simulink model "PMSMdetailTestbench"  (R2025b)
settings: Solver=ode1be  StartTime=0.0  StopTime=50  FixedStep=electricDrive.PmsmControlParams.Ts  RelTol=1e-3  EnableMultiTasking=on
PreLoadFcn:
  | PMSMSystemParams;
  | %PMSMthermalParams;
undefined symbols (not defined in the file or in its folder): electricDrive
libraries: fl_lib x91, nesl_utility x22, ee_lib x4, SimscapeFluids_lib x3, eeTransforms x2, simulink x2, batteryecm_lib x1, autolibshared x1, sdl_lib x1, eePmsmCurrentController x1, eePmsmFwController x1, eePmsmCurrentReferenceGen x1
(part 1 of 2)
CloseFcn:
  | try,close(h1_ee_pmsm_field_weakening_control),end
  | clear h1_ee_pmsm_field_weakening_control
  | 
  | clear simlogPMSMfocControlLossMaoGen
  | clear logsoutPMSMfocControlLossMaoGen
  | clear air_density alpha beta  Cdc CopperDensity CopperSpHeat CopperThconductivity Cp Cv drag_coefficient dt  gravity h h_conv IronDensity IronSpHeat IronThConductivity Jm k Ld lossMat Lq  max_power max_torque MotorThermal nu p Pmax PmsmControlParams PmsmParams rho  spMat tqMat tout T Tmax  u VehicleParams Vnom
Description:
  | Copyright 2022 - 2023 The MathWorks, Inc.
settings Model: Creator=The MathWorks, Inc.  LastModifiedBy=jjha
settings SolverCC: AlgebraicLoopSolver=TrustRegion  AutoInsertRateTranBlk=on  MaxZcPerStep=1.0
settings DataIOCC: MaxDataPoints=210000  SignalLoggingName=logsoutPMSMdetailTestbench  ReturnWorkspaceOutputsName=simoutPMSMdetailTestbench
settings OptimizationCC: ReuseModelBlockBuffer=off  LifeSpan=inf
settings DebuggingCC: UnconnectedInputMsg=warning  UnconnectedOutputMsg=warning  UnconnectedLineMsg=warning  SFUnexpectedBacktrackingDiag=warning  SFNoUnconditionalDefaultTransitionDiag=warning  SFExecutionAtInitializationDiag=none  ArithmeticOperatorsInVariantConditions=warning
settings ModelReferenceCC: EnableRefExpFcnMdlSchedulingChecks=on
settings SFSimCC: SimUseLocalCustomCode=off  CustomCodeUndefinedFunction=UseInterfaceOnly
settings RTWCC: RTWUseLocalCustomCode=off  GPUComputeCapability=3.5  DLArmComputeVersion=19.05
settings CodeAppCC: StateflowObjectComments=on
settings GRTTargetCC: TargetLangStandard=C89/C90 (ANSI)
settings ConfigComp: CovMetricSettings=dw  CovSaveCumulativeToWorkspaceVar=on  CovSaveSingleToWorkspaceVar=on  CovExternalEMLEnable=off
settings SimscapeCC: SimscapeNormalizeSystem=off  SimscapeLogType=all  SimscapeLogSimulationStatistics=on  SimscapeLogName=simlogPMSMdetailTestbench  SimscapeLogDataHistory=700000.0

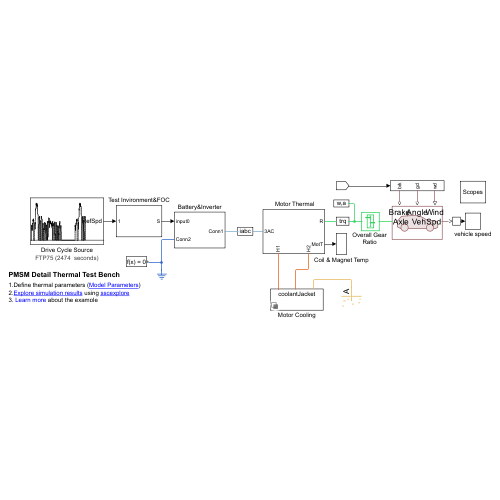
[thumbnail: Simulink's stored preview of the top-level diagram]
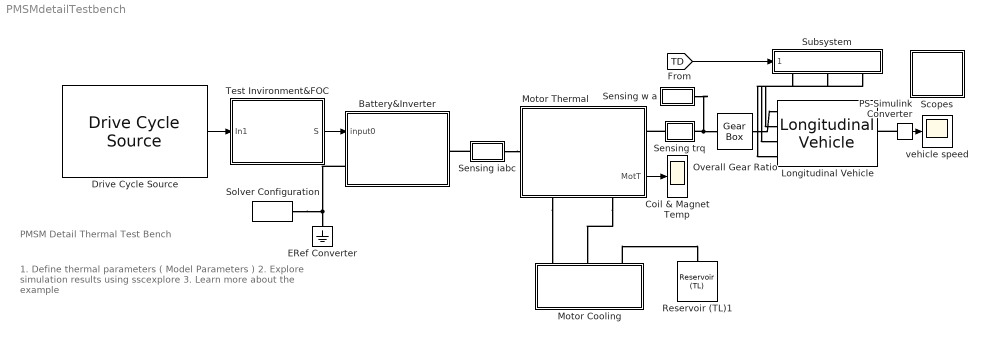
== system PMSMdetailTestbench ==
  note: PMSM Detail Thermal Test Bench
  note: 1. Define thermal parameters ( Model Parameters )
      | 2. Explore simulation results using sscexplore
      | 3. Learn more about the example
  " Motor Thermal" : Subsystem  Tag=PublishSubsystem  VariantControl=Variant1
      settings: PortSchema="{\"entries\":[{\"content\":{\"sides\":[{\"content\":{\"connectorIds\":[\"LConn1\"]},\"type\":\"ConnectorPlacement.EquallySpacedRectSide\",\"uuid\":\"590a444e-8195-4988-a9c8-7c57f93e7add\"},{\"content\":{\"connectorIds\":[\"RConn1\",\"Out1\"],\"side\":\"RIGHT\"},\"type\":\"ConnectorPlacement.EquallySpacedRectSide\",\"uuid\":\"ff30d583-60d1-4c2f-8cfa-0519d0956af2\"},{\"content\":{\"connectorIds\":[],\"side\":\"TOP\"},\"type\":\"ConnectorPlacement.EquallySpacedRectSide\",\"uuid\":\"f416ecb7-f0fa-4dcd-bce9-4bdf16786e53\"},{\"content\":{\"connectorIds\":[\"RConn2\",\"RConn3\"],\"side\":\"BOTTOM\"},\"type\":\"ConnectorPlacement.EquallySpacedRectSide\",\"uuid\":\"aeecbe3b-4b08-4b99-ab7c-25ad9565aff3\"}]},\"type\":\"ConnectorPlacement.EquallySpacedConnector\",\"uuid\":\"9ecfe474-afdb-4e00-8545-4450812d4813\"}],\"packageUris\":[\"http://schema.mathworks.com/mf0/Connector/R2020b\"],\"version\":\"1.0\"}"
  Battery&Inverter : Subsystem
  Coil & Magnet Temp : Scope
      settings: ActiveDisplayYMinimum=-45.49094  ActiveDisplayYMaximum=409.41849
  Drive Cycle Source : autolibshared/Drive Cycle Source  cycleVar=FTP75  fileVar=cycleFTP75.mat  tfinal="2474  seconds"  cycleRepeat=off  outAccPort=off  outGearPort=off  gearList=No gear data  t_wot1=5  xdot_woto=0  xdot_wot1=30  t_wot2=20  xdot_wot2=0  t_wotend=30  srcUnit=m/s  outUnit=km/hr  srcAccUnit=m/s/s  outAccUnit=m/s^2  dt=1e-3  aMode=1  faultOption=off  velBnd=2  velBndUnit=mph  inUnit=m/s  timeBnd=1  failOption=off  stopSim=off  maxFaultCnt=10  maxFaultTime=2  maxTotFaultTime=15  traceOption=off  dtTrace=1  traceWindow=10  lastDCname=FTP75  lastOutUnit=mph  lastDT=1e-3  lastTB=1  lastSB=2  forceCalcBound=off
  ERef Converter : fl_lib/Electrical/Electrical Elements/Electrical Reference
  Longitudinal Vehicle : sdl_lib/Tires & Vehicles/Longitudinal Vehicle  vehParamType=sdl.enum.VehicleParameterizationType.Regular  M_vehicle=electricDrive.VehicleParams.vehicle_mass kg  R_tireroll=electricDrive.VehicleParams.wheel_radius m  C_tireroll=electricDrive.VehicleParams.rolling_res_ratio  C_airdrag=electricDrive.drag_coefficient  A_front=electricDrive.VehicleParams.Frontalarea m^2  A_rl=120 N  B_rl=1.8 N*s/m  C_rl=0.389 N*s^2/m^2  g=electricDrive.gravity m/s^2  V_1=0.3 m/s  w_1=0.01 rad/s  ShowBrakeIn=true  ShowSlopeIn=true  SlopeInputType=sdl.enum.VehicleLongitudinalRoadSlopeInputType.Angle  ShowWindIn=true  ShowGOut=false  air_density=1.184 kg/m^3  V_x_specify=off  V_x_priority=High  V_x=0 m/s  V_x_nominal_specify=off  V_x_nominal_value=1  V_x_nominal_unit=m/s  trq_specify=off  trq_priority=None  trq=0 N*m  trq_nominal_specify=off  trq_nominal_value=1  trq_nominal_unit=N*m  w_specify=off  w_priority=None  w=0 rad/s  w_nominal_specify=off  w_nominal_value=1  w_nominal_unit=rad/s
      settings: InternalSimscapePortConfiguration="{\"Bottom\":[],\"Left\":[{\"id\":\"Axle\",\"label\":\"Axle\",\"type\":\"foundation.mechanical.rotational.rotational\"}],\"Right\":[{\"id\":\"v_out\",\"label\":\"VehSpd\",\"type\":\"output\"}],\"Top\":[{\"id\":\"brkF\",\"label\":\"Brake\",\"type\":\"input\"},{\"id\":\"angle_in\",\"label\":\"Angle\",\"type\":\"input\"},{\"id\":\"V_wind\",\"label\":\"Wind\",\"type\":\"input\"}]}"
  Motor Cooling : Subsystem  Variant=on  VariantControlMode=label  LabelModeActiveChoice=true
      settings: PortSchema="{\"entries\":[{\"content\":{\"sides\":[{\"content\":{\"connectorIds\":[]},\"type\":\"ConnectorPlacement.EquallySpacedRectSide\",\"uuid\":\"fad2e2e2-c8a8-4ae7-a5e0-e2d04801ad81\"},{\"content\":{\"connectorIds\":[],\"side\":\"RIGHT\"},\"type\":\"ConnectorPlacement.EquallySpacedRectSide\",\"uuid\":\"a876eae4-26d9-44a3-9dd3-410a35dafbf1\"},{\"content\":{\"connectorIds\":[\"LConn1\",\"LConn2\",\"LConn3\"],\"side\":\"TOP\"},\"type\":\"ConnectorPlacement.EquallySpacedRectSide\",\"uuid\":\"b2d352a8-e78b-4f23-87e4-b1c134d4f518\"}]},\"type\":\"ConnectorPlacement.EquallySpacedConnector\",\"uuid\":\"4da0a1ca-7739-4d5f-a9bc-f50bcf2d911d\"}],\"packageUris\":[\"http://schema.mathworks.com/mf0/Connector/R2020b\"],\"version\":\"1.0\"}"
  "Overall Gear Ratio " : fl_lib/Mechanical/Mechanisms/Gear Box  ratio=electricDrive.VehicleParams.Gear_ratio  t_in_specify=off  t_in_priority=High  t_in=0 N*m  t_in_nominal_specify=off  t_in_nominal_value=1  t_in_nominal_unit=N*m  t_out_specify=off  t_out_priority=High  t_out=0 N*m  t_out_nominal_specify=off  t_out_nominal_value=1  t_out_nominal_unit=N*m
  PS-Simulink Converter : nesl_utility/PS-Simulink Converter  PhysicalDomain=network_engine_domain  SubClassName=ps_output  LeftPortType=input  RightPortType=output  PseudoPeriodic=off  Frequencies=[]  VectorFormat=inherit  Unit=inherit  AffineConversion=off
  Reservoir (TL)1 : fl_lib/Thermal Liquid/Elements/Reservoir (TL)  pressure_spec=foundation.enum.pressure_spec.atmospheric  reservoir_pressure=0.101325 MPa  reservoir_temperature=293.15 K  area=0.01 m^2
  Scopes : Subsystem
      mask Display: disp(get_param(gcb,'Name'))
  Sensing w a : Subsystem
      mask Display: disp('w,a')
  Sensing iabc : Subsystem
      mask Display: disp('iabc')
  Sensing trq : Subsystem
      mask Display: disp('trq')
  Solver Configuration : nesl_utility/Solver Configuration  PhysicalDomain=network_engine_domain  SubClassName=solver  LeftPortType=input  RightPortType=generic  Tones=[]  Harmonics=[]  SimulateNoise=off  Profile=off  UseLocalSampling=off  EnableSwitchedLinearOptims=on  FrequencyDomain=off  UseCCode=off  RelTol=0.001  AbsTol=1e-06  MinStep=1e-09  ToWorkspace=off  RevertToSquareIcSolve=off  NumHomotopyIterations=100  PhasorMode=off  PhasorModeNumHarmonics=1  ConsistencySolver=NEWTON_XTOL_AFTER_FTOL  IndexReductionMethod=DerivativeReplacement  DoDC=off  ResidualTolerance=1e-9  ConsistencyTolSource=GLOBAL  ConsistencyAbsTol=0.001  ConsistencyRelTol=0.001  ConsistencyTolFactor=0.001  UseLocalSolver=on  LocalSolverChoice=NE_BACKWARD_EULER_ADVANCER  ResolveIndetEquations=on  FunctionEvalNumThread=1  LocalSolverSampleTime=electricDrive.PmsmControlParams.Ts  DoFixedCost=on  MaxNonlinIter=4  MaxModeIter=2  ComputeImpulses=off  ImpulseIterations=2  LinearAlgebra=auto  LinearAlgebraNumThread=0  EquationFormulation=NE_TIME_EF  DelaysMemoryBudget=1024  AutomaticFiltering=on  FilteringTimeConstant=0.001  PartitionStorageMethod=AS_NEEDED  PartitionMemoryBudget=1024  PartitionMethod=FAST  MultibodyUseLocalSolver=off  MultibodyLocalSolverChoice=ODE1  MultibodyLocalSolverSampleTime=0.001
  Subsystem : Subsystem
      settings: PortSchema="{\"entries\":[{\"content\":{\"sides\":[{\"content\":{\"connectorIds\":[]},\"type\":\"ConnectorPlacement.EquallySpacedRectSide\",\"uuid\":\"5b33bb33-1028-4467-9d0b-860d7c65cb16\"},{\"content\":{\"connectorIds\":[\"RConn1\",\"RConn2\",\"RConn3\"],\"side\":\"RIGHT\"},\"type\":\"ConnectorPlacement.EquallySpacedRectSide\",\"uuid\":\"d30bcb89-569c-4584-a5e8-bf96143649ac\"},{\"content\":{\"connectorIds\":[\"In1\"],\"side\":\"TOP\"},\"type\":\"ConnectorPlacement.EquallySpacedRectSide\",\"uuid\":\"a556bd16-04f6-4e3c-9a78-edea790b19fa\"}]},\"type\":\"ConnectorPlacement.EquallySpacedConnector\",\"uuid\":\"7b9502e3-af00-49d8-8813-697019fc00d4\"}],\"packageUris\":[\"http://schema.mathworks.com/mf0/Connector/R2020b\"],\"version\":\"1.0\"}"
  Test Invironment&FOC : Subsystem
  vehicle speed : Scope
      settings: ActiveDisplayYMinimum=-1.28909  ActiveDisplayYMaximum=11.51595  DataLoggingVariableName=ScopeData2
  wires:
  Drive Cycle Source/1 -> Test Invironment&FOC/1(In1)
  Test Invironment&FOC/1(S) -> Battery&Inverter/1(input0)
  [TD] -> Subsystem/1(" ")
  PS-Simulink Converter/1 -> vehicle speed/1
  " Motor Thermal"/1(MotT) -> Coil & Magnet Temp/1
  connections:
  Sensing iabc/RConn1 -- " Motor Thermal"/LConn1
  Sensing trq/LConn1 -- " Motor Thermal"/RConn1
  Sensing w a/LConn1 -- Sensing trq/RConn1 -- "Overall Gear Ratio "/LConn1
  Sensing iabc/LConn1 -- Battery&Inverter/RConn1
  Battery&Inverter/LConn1 -- Solver Configuration/RConn1 -- ERef Converter/LConn1
  Subsystem/RConn1 -- Longitudinal Vehicle/LConn2
  Subsystem/RConn2 -- Longitudinal Vehicle/LConn3
  PS-Simulink Converter/LConn1 -- Longitudinal Vehicle/RConn1
  "Overall Gear Ratio "/RConn1 -- Longitudinal Vehicle/LConn1
  Subsystem/RConn3 -- Longitudinal Vehicle/LConn4
  Motor Cooling/LConn3 -- Reservoir (TL)1/LConn1
  " Motor Thermal"/RConn3 -- Motor Cooling/LConn2
  " Motor Thermal"/RConn2 -- Motor Cooling/LConn1

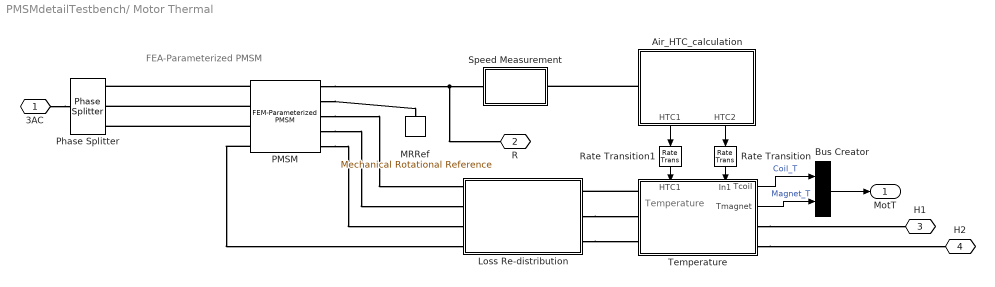
== system PMSMdetailTestbench/ Motor Thermal ==
  note: Temperature
  note: FEA-Parameterized
      | PMSM
  Air_HTC_calculation : Subsystem
      settings: PortSchema="{\"entries\":[{\"content\":{\"sides\":[{\"content\":{\"connectorIds\":[\"LConn1\"]},\"type\":\"ConnectorPlacement.EquallySpacedRectSide\",\"uuid\":\"c3fc49c2-0151-484f-b0d8-f4e4a060bcaf\"},{\"content\":{\"side\":\"RIGHT\"},\"type\":\"ConnectorPlacement.EquallySpacedRectSide\",\"uuid\":\"c73251fe-fcad-4c5f-9d27-fb7ac98c9b31\"},{\"content\":{\"side\":\"TOP\"},\"type\":\"ConnectorPlacement.EquallySpacedRectSide\",\"uuid\":\"06ea8515-c1b4-4445-9ea2-9a6fe3b8d822\"},{\"content\":{\"connectorIds\":[\"Out1\",\"Out2\"],\"side\":\"BOTTOM\"},\"type\":\"ConnectorPlacement.EquallySpacedRectSide\",\"uuid\":\"0d77474d-64a7-49ab-b2b5-eb3962b26dfa\"}]},\"type\":\"ConnectorPlacement.EquallySpacedConnector\",\"uuid\":\"651eda7a-2416-4496-9b8b-1b2d725cf6dd\"}],\"packageUris\":[\"http://schema.mathworks.com/mf0/Connector/R2020b\"],\"version\":\"1.0\"}"
  Bus Creator : BusCreator  Inputs=2
  Loss Re-distribution : Subsystem
  MRRef : fl_lib/Mechanical/Rotational Elements/Mechanical Rotational Reference
  PMSM : ee_lib/Electromechanical/Permanent Magnet/FEM-Parameterized PMSM  parameterization=1  winding_type=ee.enum.statorconnection.wye  iVec=[-2, 0, 2] A  xVec=[0, 20, 40, 60] deg  dfluxdiMatrix=0.0002 * ones(3, 4) Wb/A  dfluxdxMatrix=[0, -.16, .16, 0; 0, -.16, .16, 0; 0, -.16, .16, 0] Wb/rad  calculate_torque_matrix=1  TorqueMatrix=zeros(3, 3, 3, 4) N*m  idVec1=[-200, 0, 200] A  iqVec1=[-200, 0, 200] A  LdMatrix=0.0002 * ones(3, 3) H  LqMatrix=0.0002 * ones(3, 3) H  PmMatrix=0.1 * ones(3, 3) Wb  interp_method=simscape.enum.interpolation.linear  N=6  Rs=electricDrive.PmsmParams.StatorResistance Ohm  Ms=0.00002 H  L0=0.00016 H  loss_param=ee.enum.fem_motor.ironLossesExtended.tabulated  losses_oc=[0, 0, 0] W  losses_sc=[0, 0, 0] W  f_losses=100 % dummy value, not required Hz  Isc_losses=95 A  Inertia=electricDrive.PmsmParams.RotorInertia kg*m^2  lam=0 N*m/(rad/s)  i_d_specify=off  i_d_priority=High  i_d=0 A  i_d_nominal_specify=off  i_d_nominal_value=1  i_d_nominal_unit=A  i_q_specify=off  i_q_priority=High  i_q=0 A  i_q_nominal_specify=off  i_q_nominal_value=1  i_q_nominal_unit=A  torque_specify=off  torque_priority=None  torque=0 N*m  torque_nominal_specify=off  torque_nominal_value=1  torque_nominal_unit=N*m  angular_velocity_specify=off  angular_velocity_priority=High  angular_velocity=PmsmParams.InitialRotorSpeed_rpm rpm  angular_velocity_nominal_specify=off  angular_velocity_nominal_value=1  angular_velocity_nominal_unit=rpm  angular_position_specify=on  angular_position_priority=High  angular_position=electricDrive.PmsmParams.InitialRotorAngle_rad rad  angular_position_nominal_specify=off  angular_position_nominal_value=1  angular_position_nominal_unit=deg  alpha=0.00386 1/K  alpha_flux=-0.001 1/K  Tmeas=283.15 K  stator_thermal_mass=electricDrive.MotorThermal.PhaseWindingThMass J/K  stator_initial_temperatures=[298.15, 298.15, 298.15] K  rotor_thermal_mass=electricDrive.MotorThermal.RotorThMass J/K  rotor_initial_temperature=298.15 K  Rm_percent_rotor=90  Rd_percent_rotor=30  idVec=[-200, 0, 200] A  iqVec=[-200, 0, 200] A  dfluxAdiaMatrix3D=zeros(3, 3, 4) Wb/A  dfluxAdibMatrix3D=zeros(3, 3, 4) Wb/A  dfluxAdicMatrix3D=zeros(3, 3, 4) Wb/A  dfluxAdxMatrix3D=zeros(3, 3, 4) Wb/rad  TorqueMatrix3D=zeros(3, 3, 4) N*m  iaVec=[-200, 0, 200] A  ibVec=[-200, 0, 200] A  icVec=[-200, 0, 200] A  dfluxAdiaMatrix=zeros(3, 3, 3, 4) Wb/A  dfluxAdibMatrix=zeros(3, 3, 3, 4) Wb/A  dfluxAdicMatrix=zeros(3, 3, 3, 4) Wb/A  dfluxAdxMatrix=zeros(3, 3, 3, 4) Wb/rad  param_dq0=ee.enum.fem_motor.fluxTabulationOption.DQpolar  winding_type_dq0=ee.enum.statorconnection.wye  expose_neutral_port=ee.enum.fem_motor.exposeNeutralPort.no  nPolePairs=electricDrive.PmsmParams.NumPolePairs  parks_type=ee.enum.fem_motor.parksType.QleadsD_AphaseToQaxis  idVec2=[-200, 0, 200] A  iqVec2=[-200, 0, 200] A  magVec2=electricDrive.PmsmParams.CurrMagVec*1.3 A  betaVec2=electricDrive.PmsmParams.CurrAdvAngleVec deg  xVec2=electricDrive.PmsmParams.RotorAngleVec deg  fluxD_dq0=zeros(3, 3, 7) Wb  fluxQ_dq0=zeros(3, 3, 7) Wb  fluxA_dq0=zeros(3, 3, 7) Wb  Torque_dq0=zeros(3, 3, 7) N*m  fluxD_IBX=electricDrive.PmsmParams.FluxDMat Wb  fluxQ_IBX=electricDrive.PmsmParams.FluxQMat Wb  fluxA_IBX=fluxAmat Wb  Torque_IBX=electricDrive.PmsmParams.TorqueMat N*m  rotorLossCoeff_k_h_DQ=zeros(3, 3) W/Hz  rotorLossCoeff_k_J_DQ=zeros(3, 3) W/Hz^2  rotorLossCoeff_k_ex_DQ=zeros(3, 3) W/Hz^(3/2)  rotorLossCoeff_k_h_IB=electricDrive.PmsmParams.RotorKhMat W/Hz  rotorLossCoeff_k_J_IB=electricDrive.PmsmParams.RotorKjMat W/Hz^2  rotorLossCoeff_k_ex_IB=electricDrive.PmsmParams.RotorKexMat W/Hz^(3/2)  statorLossCoeff_k_h_DQ=zeros(3, 3) W/Hz  statorLossCoeff_k_J_DQ=zeros(3, 3) W/Hz^2  statorLossCoeff_k_ex_DQ=zeros(3, 3) W/Hz^(3/2)  statorLossCoeff_k_h_IB=electricDrive.PmsmParams.StatorKhMat W/Hz  statorLossCoeff_k_J_IB=electricDrive.PmsmParams.StatorKjMat W/Hz^2  statorLossCoeff_k_ex_IB=electricDrive.PmsmParams.StatorKexMat W/Hz^(3/2)  wVec=[1000, 2000] rpm  rotorLossTable_DQ=zeros(3, 3, 2) W  statorLossTable_DQ=zeros(3, 3, 2) W  rotorLossTable_IB=zeros(3, 5, 2) W  statorLossTable_IB=zeros(3, 5, 2) W  electrical_torque_before_iron_losses_specify=off  electrical_torque_before_iron_losses_priority=None  electrical_torque_before_iron_losses=0 N*m  electrical_torque_before_iron_losses_nominal_specify=off  electrical_torque_before_iron_losses_nominal_value=1  electrical_torque_before_iron_losses_nominal_unit=N*m  Qrotor_specify=off  Qrotor_priority=None  Qrotor=0 J/s  Qrotor_nominal_specify=off  Qrotor_nominal_value=1  Qrotor_nominal_unit=J/s  Qstator_specify=off  Qstator_priority=None  Qstator=0 J/s  Qstator_nominal_specify=off  Qstator_nominal_value=1  Qstator_nominal_unit=J/s
      settings: InternalSimscapePortConfiguration="{\"Bottom\":[],\"Left\":[{\"id\":\"a\",\"label\":\"a\",\"type\":\"foundation.electrical.electrical\"},{\"id\":\"b\",\"label\":\"b\",\"type\":\"foundation.electrical.electrical\"},{\"id\":\"c\",\"label\":\"c\",\"type\":\"foundation.electrical.electrical\"},{\"id\":\"HR\",\"label\":\"HR\",\"type\":\"foundation.thermal.thermal\"}],\"Right\":[{\"id\":\"R\",\"label\":\"R\",\"type\":\"foundation.mechanical.rotational.rotational\"},{\"id\":\"C\",\"label\":\"C\",\"type\":\"foundation.mechanical.rotational.rotational\"},{\"id\":\"HA\",\"label\":\"HA\",\"type\":\"foundation.thermal.thermal\"},{\"id\":\"HB\",\"label\":\"HB\",\"type\":\"foundation.thermal.thermal\"},{\"id\":\"HC\",\"label\":\"HC\",\"type\":\"foundation.thermal.thermal\"}],\"Top\":[]}"
  Phase Splitter : ee_lib/Connectors & References/Phase Splitter
  Rate Transition : RateTransition
  Rate Transition1 : RateTransition
  Speed Measurement : Subsystem
  Temperature : Subsystem
      settings: PortSchema="{\"entries\":[{\"content\":{\"sides\":[{\"content\":{\"connectorIds\":[\"LConn1\",\"LConn2\",\"LConn3\"]},\"type\":\"ConnectorPlacement.EquallySpacedRectSide\",\"uuid\":\"fee72484-960d-4cd4-9296-e38678962aa1\"},{\"content\":{\"connectorIds\":[\"Out1\",\"Out2\",\"RConn1\",\"RConn2\"],\"side\":\"RIGHT\"},\"type\":\"ConnectorPlacement.EquallySpacedRectSide\",\"uuid\":\"5fc115b4-63fd-47d3-871d-1c82ac52ac43\"},{\"content\":{\"connectorIds\":[\"In1\",\"In2\"],\"side\":\"TOP\"},\"type\":\"ConnectorPlacement.EquallySpacedRectSide\",\"uuid\":\"406f719a-f995-4122-9f35-24e8332a2e84\"},{\"content\":{\"connectorIds\":[],\"side\":\"BOTTOM\"},\"type\":\"ConnectorPlacement.EquallySpacedRectSide\",\"uuid\":\"14dc85e6-8157-4b38-8651-862ce77721cd\"}]},\"type\":\"ConnectorPlacement.EquallySpacedConnector\",\"uuid\":\"1dcc2b5d-90fd-40de-873d-99118eb86bdd\"}],\"packageUris\":[\"http://schema.mathworks.com/mf0/Connector/R2020b\"],\"version\":\"1.0\"}"
  3AC : PMIOPort  Side=Left
  R : PMIOPort  Port=2  Side=Right
  H1 : PMIOPort  Port=3  Side=Right
  H2 : PMIOPort  Port=4  Side=Right
  MotT : Outport
  wires:
  Temperature/2(Tmagnet) -> Bus Creator/2  "Magnet_T"
  Rate Transition/1 -> Temperature/2(In1)
  Air_HTC_calculation/2(HTC2) -> Rate Transition/1
  Air_HTC_calculation/1(HTC1) -> Rate Transition1/1
  Rate Transition1/1 -> Temperature/1(HTC1)
  Bus Creator/1 -> MotT/1
  Temperature/1(Tcoil) -> Bus Creator/1  "Coil_T"
  connections:
  PMSM/LConn2 -- Phase Splitter/RConn2
  PMSM/RConn2 -- MRRef/LConn1
  PMSM/RConn1 -- R/RConn1 -- Speed Measurement/LConn1
  PMSM/LConn1 -- Phase Splitter/RConn1
  Air_HTC_calculation/LConn1 -- Speed Measurement/RConn1
  Loss Re-distribution/RConn2 -- Temperature/LConn2
  Loss Re-distribution/RConn3 -- Temperature/LConn3
  PMSM/LConn3 -- Phase Splitter/RConn3
  PMSM/LConn4 -- Loss Re-distribution/LConn4
  PMSM/RConn3 -- Loss Re-distribution/LConn1
  PMSM/RConn4 -- Loss Re-distribution/LConn2
  PMSM/RConn5 -- Loss Re-distribution/LConn3
  3AC/RConn1 -- Phase Splitter/LConn1
  Temperature/LConn1 -- Loss Re-distribution/RConn1
  Temperature/RConn1 -- H1/RConn1
  Temperature/RConn2 -- H2/RConn1

== system PMSMdetailTestbench/Battery&Inverter ==
  input0 : Inport
  Average-Value Voltage Source Converter (Three-Phase) : ee_lib/Semiconductors & Converters/Converters/Average-Value Voltage Source Converter (Three-Phase)  port_option=ee.enum.threePhasePort.composite  frequency_option=ee.enum.converters.frequency.variable  input_option=ee.enum.converters.inputOption.ModWave  FRated=60 Hz  losses_parameterization=ee.enum.converters.losses.fixed  Pfixed=1 W  ks=0.01  kc1=1.7 V  kc2=0.01 Ohm  Ploss_vect=[100, 800, 1870, 3250, 4900] W  Irms_vect=[10, 100, 200, 300, 400] A  Vdc_nom=300 V  thermal_mass=30000 J/K  temperature_specify=off  temperature_priority=High  temperature=298.15 K  temperature_nominal_specify=off  temperature_nominal_value=1  temperature_nominal_unit=K
      settings: InternalSimscapePortConfiguration="{\"Bottom\":[],\"Left\":[{\"id\":\"ModWave\",\"label\":\"ModWave\",\"type\":\"input\"},{\"id\":\"N\",\"label\":\"~\",\"type\":\"foundation.electrical.three_phase\"}],\"Right\":[{\"id\":\"p\",\"label\":\"+\",\"type\":\"foundation.electrical.electrical\"},{\"id\":\"n\",\"label\":\"-\",\"type\":\"foundation.electrical.electrical\"}],\"Top\":[]}"
  Battery : batteryecm_lib/Battery  Vnom=electricDrive.Vnom V  prm_dir=1  R1_dis=2 Ohm  R1_ch=2 Ohm  R1=0.001 Ohm  prm_AH=simscape.enum.battery.prm_AH.infinite  AH=200 hr*A  V1=290 V  AH1=50 hr*A  prm_R2=1  R2=2000 Ohm  Tmeas=298.15 K  charge_measurement_port=simscape.enum.battery.enable.no  prm_dyn=1  Rp1=0.005 Ohm  tau1=30 s  Rp2=0.005 Ohm  tau2=30 s  Rp3=0.005 Ohm  tau3=30 s  Rp4=0.005 Ohm  tau4=30 s  Rp5=0.005 Ohm  tau5=30 s  prm_fade=1  N_fade=100  AH_fade=45 hr*A  R1_fade=2.02 Ohm  R1_ch_fade=2.02 Ohm  V1_fade=10.35 V  prm_age=1  prm_age_OCV=1  OCV_age=0.9  SOC_age=60  Tmeas_age=298.15 K  delta_time_age_vec=[0] d  temperature_age_vec=[273] K  OCV_scaling_age=2.2134e6  OCV_offset_age=1.632e6  temp_exp_age=0.515833569 V  t_exp_age=0.75  Vnom_T2=12 V  R1_T2=2.2 Ohm  R1_T2_dis=2.2 Ohm  R1_T2_ch=2.2 Ohm  V1_T2=11.4 V  R2_T2=2200 Ohm  Rp1_T2=0.005 Ohm  tau1_T2=30 s  Rp2_T2=0.005 Ohm  tau2_T2=30 s  Rp3_T2=0.005 Ohm  tau3_T2=30 s  Rp4_T2=0.005 Ohm  tau4_T2=30 s  Rp5_T2=0.005 Ohm  tau5_T2=30 s  Tmeas2=273.15 K  thermal_port=simscape.enum.thermaleffects.omit  thermal_mass=30000 J/K  i_specify=off  i_priority=None  i=0 A  i_nominal_specify=off  i_nominal_value=1  i_nominal_unit=A  v_specify=off  v_priority=None  v=0 V  v_nominal_specify=off  v_nominal_value=1  v_nominal_unit=V  charge_specify=on  charge_priority=High  charge=200 hr*A  charge_nominal_specify=off  charge_nominal_value=1  charge_nominal_unit=A*hr  num_cycles_specify=off  num_cycles_priority=High  num_cycles=0  num_cycles_nominal_specify=off  num_cycles_nominal_value=1  num_cycles_nominal_unit=1  temperature_specify=off  temperature_priority=High  temperature=298.15 K  temperature_nominal_specify=off  temperature_nominal_value=1  temperature_nominal_unit=K
  C : fl_lib/Electrical/Electrical Elements/Capacitor  c=electricDrive.Cdc F  r=1e-6 Ohm  g=0 1/Ohm  i_specify=off  i_priority=None  i=0 A  i_nominal_specify=off  i_nominal_value=1  i_nominal_unit=A  v_specify=off  v_priority=None  v=0 V  v_nominal_specify=off  v_nominal_value=1  v_nominal_unit=V  vc_specify=on  vc_priority=None  vc=electricDrive.Vnom V  vc_nominal_specify=off  vc_nominal_value=1  vc_nominal_unit=V
  Sensing Vdc : Subsystem
      mask Display: disp('vdc')
  Simulink-PS Converter : nesl_utility/Simulink-PS Converter  PhysicalDomain=network_engine_domain  SubClassName=ps_input  LeftPortType=input  RightPortType=output  PseudoPeriodic=off  Frequencies=[]  NoiseDistribution=none  NoiseParameters=[]  Unit=1  AffineConversion=off  FilteringAndDerivatives=provide  SimscapeFilterOrder=1  InputFilterTimeConstant=0.001  UdotUserProvided=0
  Conn2 : PMIOPort  Side=Left
  Conn1 : PMIOPort  Port=2  Side=Right
  wires:
  input0/1 -> Simulink-PS Converter/1
  connections:
  Conn1/RConn1 -- Average-Value Voltage Source Converter (Three-Phase)/LConn2
  Battery/RConn1 -- Average-Value Voltage Source Converter (Three-Phase)/RConn2 -- Sensing Vdc/RConn1 -- C/RConn1 -- Conn2/RConn1
  Sensing Vdc/LConn1 -- Average-Value Voltage Source Converter (Three-Phase)/RConn1 -- Battery/LConn1 -- C/LConn1
  Simulink-PS Converter/RConn1 -- Average-Value Voltage Source Converter (Three-Phase)/LConn1

== system PMSMdetailTestbench/Motor Cooling ==
  OilJet : Subsystem  VariantControl=false
  coolantJacket : Subsystem  VariantControl=true
  MHD : PMIOPort  Side=Left
  MHJ : PMIOPort  Port=2  Side=Left
  Ref : PMIOPort  Port=3  Side=Left

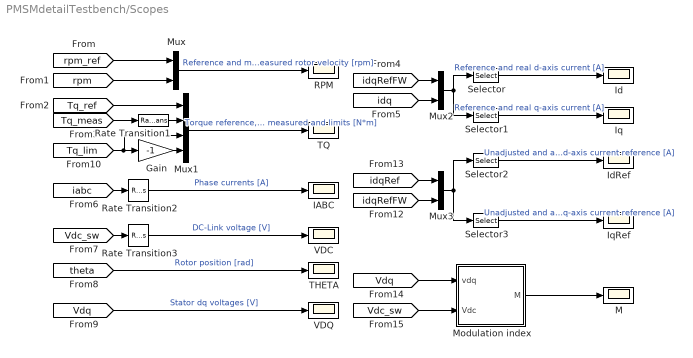
== system PMSMdetailTestbench/Scopes ==
  Gain : Gain  Gain=-1
  IABC : Scope
      settings: ActiveDisplayYMinimum=-158.01349  ActiveDisplayYMaximum=157.98632  DataLoggingSaveFormat=Array
  Id : Scope
      settings: ActiveDisplayYMinimum=-866.72955  ActiveDisplayYMaximum=3832.58854  DataLoggingVariableName=ScopeData2  DataLoggingSaveFormat=Array
  IdRef : Scope
      settings: ActiveDisplayYMinimum=-62.93355  ActiveDisplayYMaximum=6.99262  DataLoggingSaveFormat=Array
  Iq : Scope
      settings: ActiveDisplayYMinimum=-174.06811  ActiveDisplayYMaximum=31.34852  DataLoggingVariableName=ScopeData3  DataLoggingSaveFormat=Array
  IqRef : Scope
      settings: ActiveDisplayYMinimum=-26.50204  ActiveDisplayYMaximum=238.51833  DataLoggingVariableName=ScopeData2  DataLoggingSaveFormat=Array
  M : Scope
      settings: ActiveDisplayYMinimum=-0.125  ActiveDisplayYMaximum=1.125  DataLoggingSaveFormat=Array
  Modulation index : Subsystem
  Mux : Mux  Inputs=2
  Mux1 : Mux
  Mux2 : Mux  Inputs=2
  Mux3 : Mux  Inputs=2
  RPM : Scope
      settings: ActiveDisplayYMinimum=-255.1589  ActiveDisplayYMaximum=2279.13776  DataLoggingVariableName=ScopeData5  DataLoggingSaveFormat=Array
  Rate Transition1 : RateTransition
  Rate Transition2 : RateTransition  OutPortSampleTime=1e-4
  Rate Transition3 : RateTransition  OutPortSampleTime=1e-4
  Selector : Selector  InputPortWidth=4  IndexOptions=Index vector (dialog)  Indices=[1 3]  OutputSizes=1
  Selector1 : Selector  InputPortWidth=4  IndexOptions=Index vector (dialog)  Indices=[2 4]  OutputSizes=1
  Selector2 : Selector  InputPortWidth=4  IndexOptions=Index vector (dialog)  Indices=[1 3]  OutputSizes=1
  Selector3 : Selector  InputPortWidth=4  IndexOptions=Index vector (dialog)  Indices=[2 4]  OutputSizes=1
  THETA : Scope
      settings: ActiveDisplayYMinimum=-0.7854  ActiveDisplayYMaximum=7.06858  DataLoggingVariableName=ScopeData6  DataLoggingSaveFormat=Array
  TQ : Scope
      settings: ActiveDisplayYMinimum=-225.00956  ActiveDisplayYMaximum=225.00956  DataLoggingVariableName=ScopeData7  DataLoggingSaveFormat=Array
  VDC : Scope
      settings: ActiveDisplayYMinimum=-40.62138  ActiveDisplayYMaximum=365.62458  DataLoggingVariableName=ScopeData8  DataLoggingSaveFormat=Array
  VDQ : Scope
      settings: ActiveDisplayYMinimum=-210.3278  ActiveDisplayYMaximum=170.36527  DataLoggingSaveFormat=Array
  wires:
  [rpm] -> Mux/2
  Selector1/1 -> Iq/1  "Reference and real q-axis current [A]"
  Mux2/1 -> Selector1/1, Selector/1
  Gain/1 -> Mux1/4
  Rate Transition3/1 -> VDC/1  "DC-Link voltage [V]"
  [Vdc_sw] -> Rate Transition3/1
  [idqRefFW] -> Mux2/1
  [Tq_ref] -> Mux1/1
  Rate Transition2/1 -> IABC/1  "Phase currents [A]"
  [idq] -> Mux2/2
  [rpm_ref] -> Mux/1
  [iabc] -> Rate Transition2/1
  [Tq_meas] -> Rate Transition1/1
  [Vdq] -> VDQ/1  "Stator dq voltages [V]"
  Selector/1 -> Id/1  "Reference and real d-axis current [A]"
  [Tq_lim] -> Mux1/3, Gain/1
  Mux1/1 -> TQ/1  "Torque reference, measured and limits [N*m]"
  [theta] -> THETA/1  "Rotor position [rad]"
  Rate Transition1/1 -> Mux1/2
  Mux/1 -> RPM/1  "Reference and measured rotor velocity [rpm]"
  Selector2/1 -> IdRef/1  "Unadjusted and adjusted d-axis current reference [A]"
  Mux3/1 -> Selector2/1, Selector3/1
  Selector3/1 -> IqRef/1  "Unadjusted and adjusted q-axis current reference [A]"
  [idqRefFW] -> Mux3/2
  [idqRef] -> Mux3/1
  [Vdq] -> Modulation index/1(vdq)
  [Vdc_sw] -> Modulation index/2(Vdc)
  Modulation index/1(M) -> M/1

== system PMSMdetailTestbench/Sensing w a ==
  MRRef : fl_lib/Mechanical/Rotational Elements/Mechanical Rotational Reference
  Motion Sensor : fl_lib/Mechanical/Mechanical Sensors/Ideal Rotational Motion Sensor  reference=foundation.enum.MeasurementReference.difference  acceleration_port=false  velocity_port=true  position_port=true  wrap_angle=simscape.enum.onoff.off  offset=0 deg
  PS-Simulink Converter1 : nesl_utility/PS-Simulink Converter  PhysicalDomain=network_engine_domain  SubClassName=ps_output  LeftPortType=input  RightPortType=output  PseudoPeriodic=off  Frequencies=[]  VectorFormat=1-D array  Unit=rad/s  AffineConversion=off
  PS-Simulink Converter2 : nesl_utility/PS-Simulink Converter  PhysicalDomain=network_engine_domain  SubClassName=ps_output  LeftPortType=input  RightPortType=output  PseudoPeriodic=off  Frequencies=[]  VectorFormat=1-D array  Unit=rad  AffineConversion=off
  R : PMIOPort  Side=Left
  tag scope: a=global, w=global
  wires:
  PS-Simulink Converter1/1 -> [w]
  PS-Simulink Converter2/1 -> [a]
  connections:
  R/RConn1 -- Motion Sensor/LConn1
  Motion Sensor/RConn2 -- PS-Simulink Converter1/LConn1
  MRRef/LConn1 -- Motion Sensor/RConn1
  Motion Sensor/RConn3 -- PS-Simulink Converter2/LConn1

== system PMSMdetailTestbench/Sensing iabc ==
  Current Sensor : ee_lib/Sensors & Transducers/Current Sensor (Three-Phase)
  PS-Simulink Converter : nesl_utility/PS-Simulink Converter  PhysicalDomain=network_engine_domain  SubClassName=ps_output  LeftPortType=input  RightPortType=output  PseudoPeriodic=off  Frequencies=[]  VectorFormat=1-D array  Unit=A  AffineConversion=off
  1 : PMIOPort  Side=Left
  2 : PMIOPort  Port=2  Side=Right
  tag scope: iabc=global
  wires:
  PS-Simulink Converter/1 -> [iabc]
  connections:
  1/RConn1 -- Current Sensor/LConn1
  2/RConn1 -- Current Sensor/RConn2
  Current Sensor/RConn1 -- PS-Simulink Converter/LConn1

== system PMSMdetailTestbench/Sensing trq ==
  PS-Simulink Converter3 : nesl_utility/PS-Simulink Converter  PhysicalDomain=network_engine_domain  SubClassName=ps_output  LeftPortType=input  RightPortType=output  PseudoPeriodic=off  Frequencies=[]  VectorFormat=1-D array  Unit=N*m  AffineConversion=off
  Torque Sensor : fl_lib/Mechanical/Mechanical Sensors/Ideal Torque Sensor
  R : PMIOPort  Side=Left
  C : PMIOPort  Port=2  Side=Right
  tag scope: Tq_meas=global
  wires:
  PS-Simulink Converter3/1 -> [Tq_meas]
  connections:
  Torque Sensor/RConn1 -- C/RConn1
  Torque Sensor/RConn2 -- PS-Simulink Converter3/LConn1
  Torque Sensor/LConn1 -- R/RConn1

== system PMSMdetailTestbench/Subsystem ==
  " " : Inport
  Bus Selector : BusSelector  OutputSignals=Brake pedal,Incline,Wind speed
  PS Gain : fl_lib/Physical Signals/Functions/PS Gain  gain=70 N
  Simulink-PS Converter1 : nesl_utility/Simulink-PS Converter  PhysicalDomain=network_engine_domain  SubClassName=ps_input  LeftPortType=input  RightPortType=output  PseudoPeriodic=off  Frequencies=[]  NoiseDistribution=none  NoiseParameters=[]  Unit=1  AffineConversion=off  FilteringAndDerivatives=provide  SimscapeFilterOrder=1  InputFilterTimeConstant=0.001  UdotUserProvided=0
  Simulink-PS Converter2 : nesl_utility/Simulink-PS Converter  PhysicalDomain=network_engine_domain  SubClassName=ps_input  LeftPortType=input  RightPortType=output  PseudoPeriodic=off  Frequencies=[]  NoiseDistribution=none  NoiseParameters=[]  Unit=deg  AffineConversion=off  FilteringAndDerivatives=provide  SimscapeFilterOrder=1  InputFilterTimeConstant=0.001  UdotUserProvided=0
  Simulink-PS Converter3 : nesl_utility/Simulink-PS Converter  PhysicalDomain=network_engine_domain  SubClassName=ps_input  LeftPortType=input  RightPortType=output  PseudoPeriodic=off  Frequencies=[]  NoiseDistribution=none  NoiseParameters=[]  Unit=m/s  AffineConversion=off  FilteringAndDerivatives=provide  SimscapeFilterOrder=1  InputFilterTimeConstant=0.001  UdotUserProvided=0
  brk : PMIOPort  Side=Right
  gd : PMIOPort  Port=2  Side=Right
  wd : PMIOPort  Port=3  Side=Right
  wires:
  Bus Selector/2 -> Simulink-PS Converter2/1  "<Incline>"
  Bus Selector/3 -> Simulink-PS Converter3/1  "<Wind speed>"
  Bus Selector/1 -> Simulink-PS Converter1/1  "<Brake pedal>"
  " "/1 -> Bus Selector/1
  connections:
  Simulink-PS Converter2/RConn1 -- gd/RConn1
  PS Gain/RConn1 -- brk/RConn1
  Simulink-PS Converter1/RConn1 -- PS Gain/LConn1
  Simulink-PS Converter3/RConn1 -- wd/RConn1

== system PMSMdetailTestbench/Test Invironment&FOC ==
  In1 : Inport
  Field Weakning FOC Control : Subsystem
  Motor Speed Reference : Subsystem
  RT : RateTransition  OutPortSampleTime=5e-05
  Test Environment : Subsystem
  Transfer Fcn First Order : simulink/Discrete/Transfer Fcn First Order  PoleZ=0.95  ICPrevOutput=0.0  DoSatur=off
  Unit Delay : UnitDelay  SampleTime=-1  HasFrameUpgradeWarning=on
  S : Outport
  tag scope: TD=global
  wires:
  [Vdc] -> Field Weakning FOC Control/5(vdc_sens)
  In1/1 -> Unit Delay/1, RT/1
  [w] -> Field Weakning FOC Control/3(w_sens)
  [iabc] -> Field Weakning FOC Control/2(iabc_sens)
  Transfer Fcn First Order/1 -> Test Environment/1(In1)
  [a] -> Field Weakning FOC Control/4(th_sens)
  Motor Speed Reference/1(MotorSpdRef) -> Field Weakning FOC Control/1(RPMReq)
  Unit Delay/1 -> Motor Speed Reference/1(VehSpd)
  RT/1 -> Transfer Fcn First Order/1
  Test Environment/1(b) -> [TD]
  Field Weakning FOC Control/1(S) -> S/1

== system PMSMdetailTestbench/ Motor Thermal/Air_HTC_calculation ==
  Rotor side  HTC : Subsystem
  Rotor_Taylor_Couette  HTC : Subsystem
  RPM : PMIOPort  Side=Left
  HTC1 : Outport
  HTC2 : Outport  Port=2
  wires:
  Rotor side  HTC/1(Output) -> HTC2/1
  Rotor_Taylor_Couette  HTC/1(Output) -> HTC1/1
  connections:
  Rotor side  HTC/LConn1 -- RPM/RConn1 -- Rotor_Taylor_Couette  HTC/LConn1

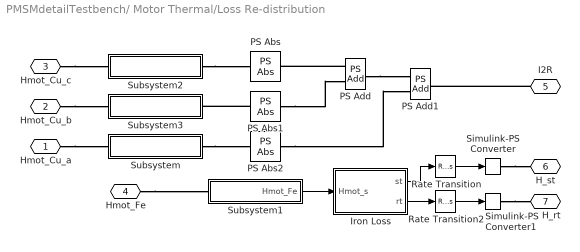
== system PMSMdetailTestbench/ Motor Thermal/Loss Re-distribution ==
  Iron Loss : Subsystem
  PS Abs : fl_lib/Physical Signals/Nonlinear Operators/PS Abs  ZeroCross=true
      settings: InternalSimscapePortConfiguration="{\"Bottom\":[],\"Left\":[{\"id\":\"I\",\"label\":\"\",\"type\":\"input\"}],\"Right\":[{\"id\":\"O\",\"label\":\"\",\"type\":\"output\"}],\"Top\":[]}"
  PS Abs1 : fl_lib/Physical Signals/Nonlinear Operators/PS Abs  ZeroCross=true
      settings: InternalSimscapePortConfiguration="{\"Bottom\":[],\"Left\":[{\"id\":\"I\",\"label\":\"\",\"type\":\"input\"}],\"Right\":[{\"id\":\"O\",\"label\":\"\",\"type\":\"output\"}],\"Top\":[]}"
  PS Abs2 : fl_lib/Physical Signals/Nonlinear Operators/PS Abs  ZeroCross=true
      settings: InternalSimscapePortConfiguration="{\"Bottom\":[],\"Left\":[{\"id\":\"I\",\"label\":\"\",\"type\":\"input\"}],\"Right\":[{\"id\":\"O\",\"label\":\"\",\"type\":\"output\"}],\"Top\":[]}"
  PS Add : fl_lib/Physical Signals/Functions/PS Add
  PS Add1 : fl_lib/Physical Signals/Functions/PS Add
  Rate Transition : RateTransition
  Rate Transition2 : RateTransition
  Simulink-PS Converter : nesl_utility/Simulink-PS Converter  PhysicalDomain=network_engine_domain  SubClassName=ps_input  LeftPortType=input  RightPortType=output  PseudoPeriodic=off  Frequencies=[]  NoiseDistribution=none  NoiseParameters=[]  Unit=W  AffineConversion=off  FilteringAndDerivatives=provide  SimscapeFilterOrder=1  InputFilterTimeConstant=0.001  UdotUserProvided=0
  Simulink-PS Converter1 : nesl_utility/Simulink-PS Converter  PhysicalDomain=network_engine_domain  SubClassName=ps_input  LeftPortType=input  RightPortType=output  PseudoPeriodic=off  Frequencies=[]  NoiseDistribution=none  NoiseParameters=[]  Unit=W  AffineConversion=off  FilteringAndDerivatives=provide  SimscapeFilterOrder=1  InputFilterTimeConstant=0.001  UdotUserProvided=0
  Subsystem : Subsystem
  Subsystem1 : Subsystem
  Subsystem2 : Subsystem
  Subsystem3 : Subsystem
  Hmot_Cu_a : PMIOPort  Side=Left
  Hmot_Cu_b : PMIOPort  Port=2  Side=Left
  Hmot_Cu_c : PMIOPort  Port=3  Side=Left
  Hmot_Fe : PMIOPort  Port=4  Side=Left
  I2R : PMIOPort  Port=5  Side=Right
  H_st : PMIOPort  Port=6  Side=Right
  H_rt : PMIOPort  Port=7  Side=Right
  wires:
  Subsystem1/1(Hmot_Fe) -> Iron Loss/1(Hmot_s)
  Iron Loss/1(st) -> Rate Transition/1
  Rate Transition/1 -> Simulink-PS Converter/1
  Iron Loss/2(rt) -> Rate Transition2/1
  Rate Transition2/1 -> Simulink-PS Converter1/1
  connections:
  Simulink-PS Converter/RConn1 -- H_st/RConn1
  Simulink-PS Converter1/RConn1 -- H_rt/RConn1
  Hmot_Cu_a/RConn1 -- Subsystem/LConn1
  Hmot_Fe/RConn1 -- Subsystem1/LConn1
  Hmot_Cu_c/RConn1 -- Subsystem2/LConn1
  Hmot_Cu_b/RConn1 -- Subsystem3/LConn1
  Subsystem2/RConn1 -- PS Abs/LConn1
  PS Abs1/LConn1 -- Subsystem3/RConn1
  PS Add/LConn1 -- PS Abs/RConn1
  PS Abs1/RConn1 -- PS Add/LConn2
  Subsystem/RConn1 -- PS Abs2/LConn1
  PS Add/RConn1 -- PS Add1/LConn1
  PS Abs2/RConn1 -- PS Add1/LConn2
  I2R/RConn1 -- PS Add1/RConn1

== system PMSMdetailTestbench/ Motor Thermal/Speed Measurement ==
  Ideal Rotational Motion Sensor : fl_lib/Mechanical/Mechanical Sensors/Ideal Rotational Motion Sensor  reference=foundation.enum.MeasurementReference.difference  acceleration_port=false  velocity_port=true  position_port=true  wrap_angle=false  offset=0 rad
  MRRef1 : fl_lib/Mechanical/Rotational Elements/Mechanical Rotational Reference
  spd : PMIOPort  Side=Right
  mot : PMIOPort  Port=2  Side=Left
  connections:
  MRRef1/LConn1 -- Ideal Rotational Motion Sensor/RConn1
  mot/RConn1 -- Ideal Rotational Motion Sensor/LConn1
  spd/RConn1 -- Ideal Rotational Motion Sensor/RConn2

== system PMSMdetailTestbench/ Motor Thermal/Temperature ==
  HTC1 : Inport
  In1 : Inport  Port=2
  PS-Simulink Converter : nesl_utility/PS-Simulink Converter  PhysicalDomain=network_engine_domain  SubClassName=ps_output  LeftPortType=input  RightPortType=output  PseudoPeriodic=off  Frequencies=[]  VectorFormat=inherit  Unit=inherit  AffineConversion=off
  Rotor Thermal Block : Subsystem
      settings: PortSchema="{\"entries\":[{\"content\":{\"sides\":[{\"content\":{\"connectorIds\":[\"Out1\"]},\"type\":\"ConnectorPlacement.EquallySpacedRectSide\",\"uuid\":\"a0a486ff-95e2-43b7-8e3c-0cd0a05f759b\"},{\"content\":{\"connectorIds\":[\"RConn1\",\"In1\",\"In2\"],\"side\":\"RIGHT\"},\"type\":\"ConnectorPlacement.EquallySpacedRectSide\",\"uuid\":\"7508b6f9-91f5-4797-b9a6-d16ad4f8253e\"},{\"content\":{\"connectorIds\":[],\"side\":\"TOP\"},\"type\":\"ConnectorPlacement.EquallySpacedRectSide\",\"uuid\":\"355558a4-f3bc-4897-a0c1-c168a45c32e0\"}]},\"type\":\"ConnectorPlacement.EquallySpacedConnector\",\"uuid\":\"a4aa0448-6fcb-4f55-be65-0b704c3933ab\"}],\"packageUris\":[\"http://schema.mathworks.com/mf0/Connector/R2020b\"],\"version\":\"1.0\"}"
  Stator Thermal Block1 : Subsystem
  I2r_loss : PMIOPort  Side=Left
  H_rt : PMIOPort  Port=2  Side=Left
  H_st : PMIOPort  Port=3  Side=Left
  H1 : PMIOPort  Port=4  Side=Right
  H2 : PMIOPort  Port=5  Side=Right
  Tcoil : Outport
  Tmagnet : Outport  Port=2
  wires:
  Rotor Thermal Block/1(mt) -> Tmagnet/1
  In1/1 -> Rotor Thermal Block/1(htc1)
  HTC1/1 -> Rotor Thermal Block/2(htc2)
  PS-Simulink Converter/1 -> Tcoil/1
  connections:
  Stator Thermal Block1/LConn1 -- PS-Simulink Converter/LConn1
  H_rt/RConn1 -- Rotor Thermal Block/RConn1
  Stator Thermal Block1/RConn1 -- H_st/RConn1
  I2r_loss/RConn1 -- Stator Thermal Block1/RConn2
  H1/RConn1 -- Stator Thermal Block1/LConn2
  H2/RConn1 -- Stator Thermal Block1/LConn3

== system PMSMdetailTestbench/Battery&Inverter/Sensing Vdc ==
  PS-Simulink Converter4 : nesl_utility/PS-Simulink Converter  PhysicalDomain=network_engine_domain  SubClassName=ps_output  LeftPortType=input  RightPortType=output  PseudoPeriodic=off  Frequencies=[]  VectorFormat=1-D array  Unit=V  AffineConversion=off
  Voltage Sensor : fl_lib/Electrical/Electrical Sensors/Voltage Sensor
  + : PMIOPort  Side=Left
  - : PMIOPort  Port=2  Side=Right
  tag scope: Vdc=global
  wires:
  PS-Simulink Converter4/1 -> [Vdc]
  connections:
  Voltage Sensor/LConn1 -- +/RConn1
  Voltage Sensor/RConn2 -- -/RConn1
  PS-Simulink Converter4/LConn1 -- Voltage Sensor/RConn1

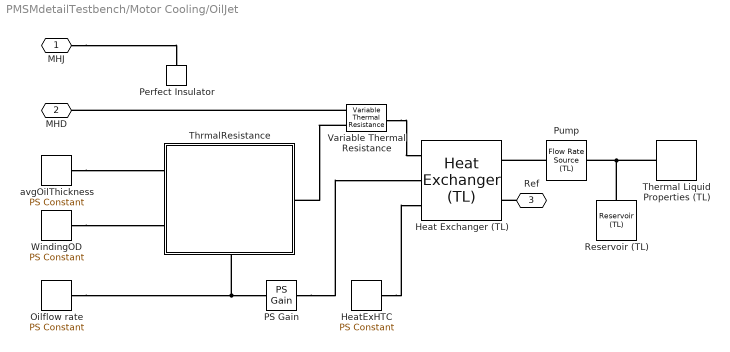
== system PMSMdetailTestbench/Motor Cooling/OilJet ==
  " Oilflow rate " : fl_lib/Physical Signals/Sources/PS Constant  constant=5/60000 m^3/s
  Heat Exchanger (TL) : SimscapeFluids_lib/Heat Exchangers/Thermal Liquid/Heat Exchanger (TL)  hex_type=fluids.heat_exchangers.enum.FlowArrangement.ParallelCounter  shell_num=1  cross_type=fluids.heat_exchangers.enum.CrossFlowArrangementTL.MixedMixed  NTU_TLU=[.5, 1, 2, 3, 4, 5]  CR_TLU=[0, .25, .5, .75, 1]  eff_TLU=[.3, .3, .3, .3, .3; .6, .55, .5, .47, .43; .85, .76, .68, .61, .55; .94, .83, .72, .65, .58; .98, .86, .75, .66, .58; .99, .86, .75, .66, .58]  R_wall=1.6e-4 K/W  min_flow_area_1=0.01 m^2  Dh_press_1=0.1 m  liquid_volume_1=0.01 m^3  Re_lam_1=2000  Re_tur_1=4000  pressure_loss_spec_1=fluids.heat_exchangers.enum.PressureLossSpec.LossCoeff  pressure_loss_coeff_1=0.1  length_press_1=1 m  length_add_1=0.1 m  roughness_1=15e-6 m  Re_friction_TLU_1=[400, 1000, 1500, 3000, 4000, 6000, 10000, 20000, 40000, 60000, 100000, 100000000]  friction_factor_TLU_1=[.264, .112, .071, .0417, .0387, .0268, .025, .0232, .0226, .022, .0214, .0214]  shape_factor_1=64  Re_Euler_TLU_1=[50, 500, 1000, 2000]  Euler_TLU_1=[4.4505, .6864, .4791, .3755]  heat_transfer_spec_1=fluids.heat_exchangers.enum.HeatCoeffSpec.Constant  heat_transfer_area_1=0.4 m^2  heat_coeff_1=250 W/(K*m^2)  length_heat_1=1 m  Nu_lam_1=3.66  Re_Colburn_TLU_1=[100, 150, 1000]  Colburn_factor_TLU_1=[.019, .013, .002]  Re_Nu_TLU_1=[100, 150, 1000]  Pr_Nu_TLU_1=[1, 10]  Nu_TLU_1=[3.72, 4.21; 3.75, 4.44; 4.21, 7.15]  fouling_factor_1=1e-4 K*m^2/W  min_heat_coeff_1=5 W/(K*m^2)  heat_transfer_area_2=0.4 m^2  fouling_factor_2=1e-4 K*m^2/W  min_heat_coeff_2=5 W/(K*m^2)  dynamic_compressibility_1=simscape.enum.onoff.on  T0_1=298.15 K  p0_1=0.101325 MPa
      settings: InternalSimscapePortConfiguration="{\"Bottom\":[],\"Left\":[{\"id\":\"A1\",\"label\":\"A1\",\"type\":\"foundation.thermal_liquid.thermal_liquid\"},{\"id\":\"B1\",\"label\":\"B1\",\"type\":\"foundation.thermal_liquid.thermal_liquid\"}],\"Right\":[{\"id\":\"H2\",\"label\":\"H2\",\"type\":\"foundation.thermal.thermal\"},{\"id\":\"C2\",\"label\":\"C2\",\"type\":\"input\"},{\"id\":\"HC2\",\"label\":\"HC2\",\"type\":\"input\"}],\"Top\":[]}"
  HeatExHTC : fl_lib/Physical Signals/Sources/PS Constant  constant=300 W/(m^2*K)
  PS Gain : fl_lib/Physical Signals/Functions/PS Gain  gain=850*2150 J/(K*m^3)
  Perfect Insulator : fl_lib/Thermal/Thermal Elements/Perfect Insulator  T_specify=off  T_priority=None  T=293.15 K  T_nominal_specify=off  T_nominal_value=1  T_nominal_unit=K
  Pump : fl_lib/Thermal Liquid/Sources/Flow Rate Source (TL)  source_type=foundation.enum.constant_controlled.constant  flow_type=foundation.enum.mass_volumetric_flow.mass  mass_flow=0.065 kg/s  volumetric_flow=0 m^3/s  power_spec=foundation.enum.power_spec.isentropic  area=pi*20^2 mm^2
      settings: InternalSimscapePortConfiguration="{\"Bottom\":[],\"Left\":[{\"id\":\"A\",\"label\":\"A\",\"type\":\"foundation.thermal_liquid.thermal_liquid\"}],\"Right\":[{\"id\":\"B\",\"label\":\"B\",\"type\":\"foundation.thermal_liquid.thermal_liquid\"}],\"Top\":[]}"
  Reservoir (TL) : fl_lib/Thermal Liquid/Elements/Reservoir (TL)  pressure_spec=foundation.enum.pressure_spec.atmospheric  reservoir_pressure=0.101325 MPa  reservoir_temperature=323.15 K  area=0.01 m^2
  Thermal Liquid Properties (TL) : SimscapeFluids_lib/Thermal Liquid/Utilities/Thermal Liquid Properties (TL)  fluid_list=fluids.thermal_liquid.utilities.enum.thermal_liquid_fluid_list.ethylene_glycol  concentration_param_EG=fluids.thermal_liquid.utilities.enum.thermal_liquid_concentration.volume_fraction  concentration_param_PG=fluids.thermal_liquid.utilities.enum.thermal_liquid_concentration.volume_fraction  c_mass_SW=3.5e-3  c_mass_EG=0.1  c_mass_PG=0.1  c_mass_GL=0.1  c_vol_EG=0.5  c_vol_PG=0.1  beta_const_EG=2.1791 GPa  beta_const_PG=2.1791 GPa  beta_const_GL=2.1791 GPa  p_min_EG=0.01 MPa  p_min_PG=0.01 MPa  p_min_GL=0.01 MPa  p_max_EG=50 MPa  p_max_PG=50 MPa  p_max_GL=50 MPa  p_atm=0.101325 MPa  properties_range_check=simscape.enum.assert.action.error
  "ThrmalResistance " : Subsystem
      settings: PortSchema="{\"entries\":[{\"content\":{\"sides\":[{\"content\":{\"connectorIds\":[\"LConn1\",\"LConn2\"]},\"type\":\"ConnectorPlacement.EquallySpacedRectSide\",\"uuid\":\"baf5ff6f-2bbb-4e60-9dad-e00baf500c6c\"},{\"content\":{\"connectorIds\":[\"RConn1\"],\"side\":\"RIGHT\"},\"type\":\"ConnectorPlacement.EquallySpacedRectSide\",\"uuid\":\"04d231ab-fa8a-490b-9fb3-01902b632b73\"},{\"content\":{\"connectorIds\":[],\"side\":\"TOP\"},\"type\":\"ConnectorPlacement.EquallySpacedRectSide\",\"uuid\":\"736d11d8-afee-4ef0-b7ea-8bcbaef6669b\"},{\"content\":{\"connectorIds\":[\"RConn2\"],\"side\":\"BOTTOM\"},\"type\":\"ConnectorPlacement.EquallySpacedRectSide\",\"uuid\":\"7a09df8f-6346-484c-a8dd-3bdb74e2d22a\"}]},\"type\":\"ConnectorPlacement.EquallySpacedConnector\",\"uuid\":\"2b9b3d82-05b9-4b26-bdd0-141d56066ae3\"}],\"packageUris\":[\"http://schema.mathworks.com/mf0/Connector/R2020b\"],\"version\":\"1.0\"}"
  Variable Thermal Resistance : fl_lib/Thermal/Thermal Elements/Variable Thermal Resistance  R_min=0 K/W  T_specify=off  T_priority=None  T=0 K  T_nominal_specify=off  T_nominal_value=1  T_nominal_unit=K  Q_specify=off  Q_priority=None  Q=0 W  Q_nominal_specify=off  Q_nominal_value=1  Q_nominal_unit=W
      settings: InternalSimscapePortConfiguration="{\"Bottom\":[],\"Left\":[{\"id\":\"A\",\"label\":\"A\",\"type\":\"foundation.thermal.thermal\"},{\"id\":\"R\",\"label\":\"R\",\"type\":\"input\"}],\"Right\":[{\"id\":\"B\",\"label\":\"B\",\"type\":\"foundation.thermal.thermal\"}],\"Top\":[]}"
  WindingOD : fl_lib/Physical Signals/Sources/PS Constant  constant=electricDrive.MotorThermal.ODpcd*1e-3 m
  avgOilThickness : fl_lib/Physical Signals/Sources/PS Constant  constant=electricDrive.MotorThermal.Oft*1e-3 m
  MHJ : PMIOPort  Side=Left
  MHD : PMIOPort  Port=2  Side=Left
  Ref : PMIOPort  Port=3  Side=Left
  connections:
  Variable Thermal Resistance/RConn1 -- Heat Exchanger (TL)/RConn1
  Variable Thermal Resistance/LConn1 -- MHD/RConn1
  " Oilflow rate "/RConn1 -- "ThrmalResistance "/RConn2 -- PS Gain/LConn1
  avgOilThickness/RConn1 -- "ThrmalResistance "/LConn1
  WindingOD/RConn1 -- "ThrmalResistance "/LConn2
  Variable Thermal Resistance/LConn2 -- "ThrmalResistance "/RConn1
  Ref/RConn1 -- Heat Exchanger (TL)/LConn2
  Reservoir (TL)/LConn1 -- Thermal Liquid Properties (TL)/RConn1 -- Pump/LConn1
  Pump/RConn1 -- Heat Exchanger (TL)/LConn1
  HeatExHTC/RConn1 -- Heat Exchanger (TL)/RConn3
  PS Gain/RConn1 -- Heat Exchanger (TL)/RConn2
  MHJ/RConn1 -- Perfect Insulator/LConn1

== system PMSMdetailTestbench/Motor Cooling/coolantJacket ==
  Perfect Insulator : fl_lib/Thermal/Thermal Elements/Perfect Insulator  T_specify=off  T_priority=None  T=293.15 K  T_nominal_specify=off  T_nominal_value=1  T_nominal_unit=K
  Pipe : fl_lib/Thermal Liquid/Elements/Pipe (TL)  length=electricDrive.MotorThermal.ChannelLength mm  area=electricDrive.MotorThermal.ChannelSection mm^2  Dh=electricDrive.MotorThermal.ChannelHydraulicdia mm  length_add=500 mm  roughness=1.5e-5 m  Re_lam=2e+3  Re_tur=4e+3  shape_factor=64  Nu_lam=3.66  dynamic_compressibility=1  inertia=0  p0=1.1 atm  T0=298.15 K  mdot0=0.1 kg/s  p_nominal=0.101325 MPa  T_nominal=293.15 K
  Pump : fl_lib/Thermal Liquid/Sources/Flow Rate Source (TL)  source_type=foundation.enum.constant_controlled.constant  flow_type=foundation.enum.mass_volumetric_flow.mass  mass_flow=0.065 kg/s  volumetric_flow=0 m^3/s  power_spec=foundation.enum.power_spec.isentropic  area=pi*20^2 mm^2
      settings: InternalSimscapePortConfiguration="{\"Bottom\":[],\"Left\":[{\"id\":\"A\",\"label\":\"A\",\"type\":\"foundation.thermal_liquid.thermal_liquid\"}],\"Right\":[{\"id\":\"B\",\"label\":\"B\",\"type\":\"foundation.thermal_liquid.thermal_liquid\"}],\"Top\":[]}"
  Reservoir (TL) : fl_lib/Thermal Liquid/Elements/Reservoir (TL)  pressure_spec=foundation.enum.pressure_spec.atmospheric  reservoir_pressure=0.101325 MPa  reservoir_temperature=298.15 K  area=0.01 m^2
  Thermal Liquid Properties (TL) : SimscapeFluids_lib/Thermal Liquid/Utilities/Thermal Liquid Properties (TL)  fluid_list=fluids.thermal_liquid.utilities.enum.thermal_liquid_fluid_list.ethylene_glycol  concentration_param_EG=fluids.thermal_liquid.utilities.enum.thermal_liquid_concentration.volume_fraction  concentration_param_PG=fluids.thermal_liquid.utilities.enum.thermal_liquid_concentration.volume_fraction  c_mass_SW=3.5e-3  c_mass_EG=0.1  c_mass_PG=0.1  c_mass_GL=0.1  c_vol_EG=0.5  c_vol_PG=0.1  beta_const_EG=2.1791 GPa  beta_const_PG=2.1791 GPa  beta_const_GL=2.1791 GPa  p_min_EG=0.01 MPa  p_min_PG=0.01 MPa  p_min_GL=0.01 MPa  p_max_EG=50 MPa  p_max_PG=50 MPa  p_max_GL=50 MPa  p_atm=0.101325 MPa  properties_range_check=simscape.enum.assert.action.error
  MHJ : PMIOPort  Side=Left
  MHD : PMIOPort  Port=2  Side=Left
  Ref : PMIOPort  Port=3  Side=Left
  connections:
  Reservoir (TL)/LConn1 -- Thermal Liquid Properties (TL)/RConn1 -- Pump/LConn1
  Pipe/LConn2 -- MHJ/RConn1
  Pipe/RConn1 -- Pump/RConn1
  Pipe/LConn1 -- Ref/RConn1
  MHD/RConn1 -- Perfect Insulator/LConn1
